simulink model "Khaled_Quantizer_Model"  (R2026b)
settings: Solver=FixedStepDiscrete  StopTime=tEnd  FixedStep=1/Fs
undefined symbols (not defined in the file): Bsim, Fs
settings Model: Creator=Maarouf  LastModifiedBy=Maarouf

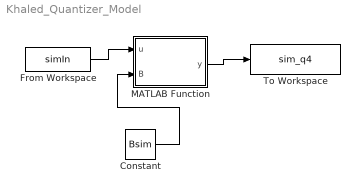
== system Khaled_Quantizer_Model ==
  Constant : Constant  Value=Bsim
  From Workspace : FromWorkspace  VariableName=simIn  SampleTime=1/Fs  Interpolate=off  OutputAfterFinalValue=Holding final value
  MATLAB Function : MATLAB Function  TreatAsAtomicUnit=on
  To Workspace : ToWorkspace  VariableName=sim_q4  SaveFormat=Timeseries  SampleTime=-1
  wires:
  From Workspace/1 -> MATLAB Function/1(u)
  MATLAB Function/1(y) -> To Workspace/1
  Constant/1 -> MATLAB Function/2(B)

== matlab function Khaled_Quantizer_Model/MATLAB Function ==
  data: u input; y output; B input

function y = fcn(u, B)
% Uniform signed audio quantizer
% u = input audio sample
% B = effective bit depth

% Preserve the unchanged 16-bit reference
if B == 16
    y = u;
else
    % Uniform quantization step
    delta = 2 / (2^B);

    % Convert sample to integer index
    index = round(u / delta);

    % Apply clipping
    minIndex = -2^(B-1);
    maxIndex = 2^(B-1) - 1;

    index = min(max(index, minIndex), maxIndex);

    % Convert back to amplitude
    y = index * delta;
end

end
